simulink model "jones_chopper"  (R2021a)
settings: Solver=VariableStepAuto  StartTime=0.0  StopTime=0.08  RelTol=1e-3
libraries: spsSeriesRLCBranchLib x3, spsDiodeLib x2, spsMeanLib x2, spsThyristorLib x2, spsVoltageMeasurementLib x2, spsCurrentMeasurementLib x1, spsDCVoltageSourceLib x1, spspowerguiLib x1
settings Model: Creator=lenovo  LastModifiedBy=lenovo

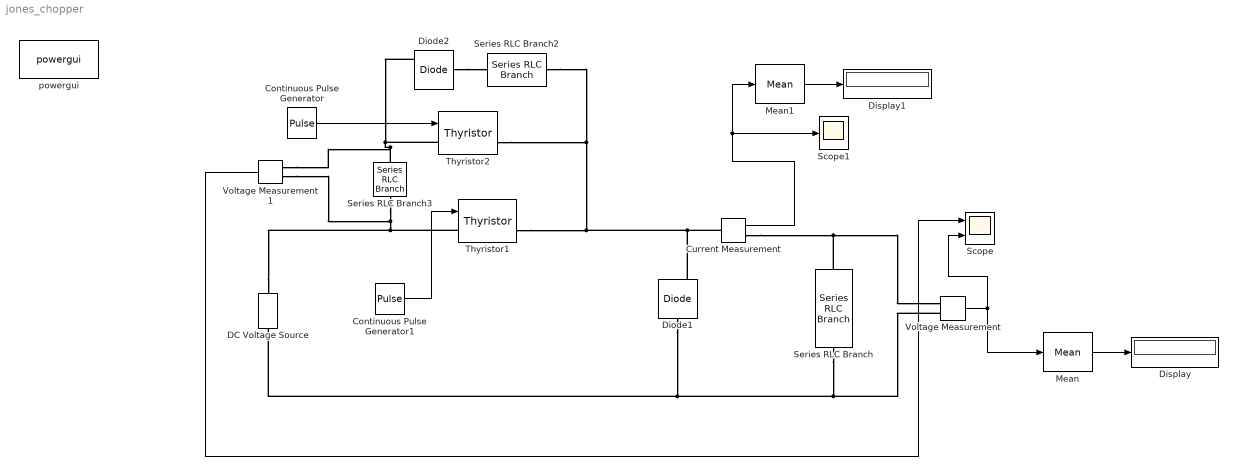
== system jones_chopper ==
  Continuous Pulse Generator : DiscretePulseGenerator  PulseType=Time based  Period=0.01  PulseWidth=50  PhaseDelay=0.005
  Continuous Pulse Generator1 : DiscretePulseGenerator  PulseType=Time based  Period=0.01  PulseWidth=50
  Current Measurement : spsCurrentMeasurementLib/Current Measurement  PhasorSimulation=off  OutputType=Complex  PSBequivalent=0
  DC Voltage Source : spsDCVoltageSourceLib/DC Voltage Source  Amplitude=120  Measurements=None
  Diode1 : spsDiodeLib/Diode  Ron=0.001  Lon=0  Vf=0.8  IC=0  UseSnubber=0  Rs=500  Cs=250e-9  Measurements=on
  Diode2 : spsDiodeLib/Diode  Ron=0.001  Lon=0  Vf=0.8  IC=0  UseSnubber=0  Rs=500  Cs=250e-9  Measurements=on
  Display : Display
  Display1 : Display
  Mean : spsMeanLib/Mean  Freq=60  Vinit=0  Ts=0
  Mean1 : spsMeanLib/Mean  Freq=60  Vinit=0  Ts=0
  Scope : Scope  NumInputPorts=2
  Scope1 : Scope
  Series RLC Branch : spsSeriesRLCBranchLib/Series RLC Branch  LConnTagsString=__new0  RConnTagsString=__new0  BranchType=RL  Resistance=30.6  Inductance=44e-3  SetiL0=off  InitialCurrent=0  Capacitance=1e-6  Setx0=off  InitialVoltage=0  Measurements=None
  Series RLC Branch2 : spsSeriesRLCBranchLib/Series RLC Branch  LConnTagsString=__new0  RConnTagsString=__new0  BranchType=L  Resistance=1  Inductance=75e-6  SetiL0=off  InitialCurrent=0  Capacitance=1e-6  Setx0=off  InitialVoltage=0  Measurements=None
  Series RLC Branch3 : spsSeriesRLCBranchLib/Series RLC Branch  LConnTagsString=__new0  RConnTagsString=__new0  BranchType=C  Resistance=1  Inductance=1e-3  SetiL0=off  InitialCurrent=0  Capacitance=8e-6  Setx0=on  InitialVoltage=120  Measurements=None
  Thyristor1 : spsThyristorLib/Thyristor  Ron=0.001  Lon=0  Vf=0.8  IC=0  Rs=500  Cs=250e-9  Measurements=on
  Thyristor2 : spsThyristorLib/Thyristor  Ron=0.001  Lon=0  Vf=0.8  IC=0  Rs=500  Cs=250e-9  Measurements=on
  Voltage Measurement : spsVoltageMeasurementLib/Voltage Measurement  PhasorSimulation=off  OutputType=Complex  PSBequivalent=0
  Voltage Measurement1 : spsVoltageMeasurementLib/Voltage Measurement  PhasorSimulation=off  OutputType=Complex  PSBequivalent=0
  powergui : spspowerguiLib/powergui  Priority=1  SimulationMode=Continuous  SampleTime=50e-6  frequency=60  Iterations=50  frequencyindice=0  Pbase=100e6  ErrMax=1e-4  UnitsV=kV  UnitsW=MW  buscounter=0  FunctionMessages=off  echomessages=off  EnableUseOfTLC=off  CurrentSourceSwitches=off  DisableSnubberDevices=off  DisableRonSwitches=off  DisableVfSwitches=off  DisplayEquations=off  AutomaticDiscreteSolvers=off  SolverType=Tustin/Backward Euler (TBE)  Interpol=off  ExternalGateDelay=off  methode=off  Ts=100  x0status=blocks  SPID=on  SwTol=0  HookPort=off  NonlinearTolerance=1e-4  nMaxIteration=100  ContinueOnMaxIteration=off  RestoreLinks=warning  ResistiveCurrentMeasurement=off  Frange=[0:2:500]  Ylog=off  Xlog=on  ShowGrid=off  save=off  variable=ZData  structure=0  ZoomFFT=off  StartTime=0.0  cycles=1  DisplayStyle=1  fundamental=60  FreqAxis=off  MaxFrequency=1000  frequencyindicesteady=1  RmsSteady=1  display=off
  wires:
  Mean/1 -> Display/1
  Mean1/1 -> Display1/1
  Current Measurement/1 -> Mean1/1, Scope1/1
  Voltage Measurement/1 -> Mean/1, Scope/2
  Continuous Pulse Generator1/1 -> Thyristor1/1
  Continuous Pulse Generator/1 -> Thyristor2/1
  Voltage Measurement1/1 -> Scope/1
  connections:
  DC Voltage Source/RConn1 -- Thyristor1/LConn1 -- Voltage Measurement1/LConn1 -- Series RLC Branch3/LConn1
  Thyristor2/RConn1 -- Series RLC Branch2/LConn1 -- Thyristor1/RConn1 -- Diode1/RConn1 -- Current Measurement/LConn1
  DC Voltage Source/LConn1 -- Diode1/LConn1 -- Voltage Measurement/LConn2 -- Series RLC Branch/RConn1
  Series RLC Branch3/RConn1 -- Voltage Measurement1/LConn2 -- Diode2/RConn1 -- Thyristor2/LConn1
  Diode2/LConn1 -- Series RLC Branch2/RConn1
  Series RLC Branch/LConn1 -- Current Measurement/RConn1 -- Voltage Measurement/LConn1
